simulink model "FilterLib_Test"  (R2018a)
settings: Solver=FixedStepDiscrete  StartTime=0.0  StopTime=5  FixedStep=Ts_task  RelTol=1e-3
PreLoadFcn:
  | Ts_task = 0.001;
InitFcn:
  | if ~exist('Ts_task','var'), Ts_task = 0.001; end
libraries: FilterLib x4
settings Model: Creator=Ismail Shaikh  LastModifiedBy=Ismail Shaikh

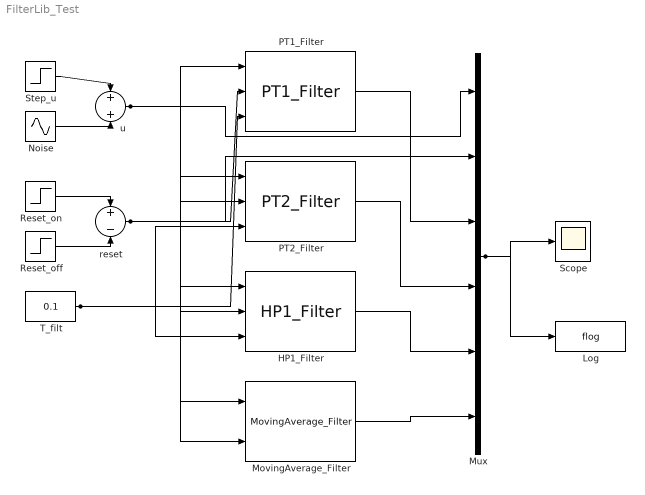
== system FilterLib_Test ==
  HP1_Filter : FilterLib/HP1_Filter  Ts=Ts_task  Method=Exact: K = 1-exp(-Ts/T)  y0=0
      settings: SourceProductName=Filter Library
  Log : ToWorkspace  VariableName=flog  SaveFormat=Structure With Time  SampleTime=-1
  MovingAverage_Filter : FilterLib/MovingAverage_Filter  N=20  y0=0
      settings: SourceProductName=Filter Library
  Mux : Mux  Inputs=6
  Noise : Sin  Amplitude=0.2  Frequency=2*pi*50  SampleTime=Ts_task
  PT1_Filter : FilterLib/PT1_Filter  Ts=Ts_task  Method=Exact: K = 1-exp(-Ts/T)  y0=0
      settings: SourceProductName=Filter Library
  PT2_Filter : FilterLib/PT2_Filter  Ts=Ts_task  Method=Exact: K = 1-exp(-Ts/T)  y0=0
      settings: SourceProductName=Filter Library
  Reset_off : Step  Time=3.05  SampleTime=Ts_task
  Reset_on : Step  Time=3  SampleTime=Ts_task
  Scope : Scope
  Step_u : Step  Time=0.5  SampleTime=Ts_task
  T_filt : Constant  Value=0.1
  reset : Sum  Inputs=+-
  u : Sum
  wires:
  Step_u/1 -> u/1
  Noise/1 -> u/2
  Reset_on/1 -> reset/1
  Reset_off/1 -> reset/2
  u/1 -> PT1_Filter/1, PT2_Filter/1, HP1_Filter/1, MovingAverage_Filter/1, Mux/1
  reset/1 -> PT1_Filter/2, PT2_Filter/2, HP1_Filter/2, MovingAverage_Filter/2, Mux/2
  T_filt/1 -> PT1_Filter/3, PT2_Filter/3, HP1_Filter/3
  PT1_Filter/1 -> Mux/3
  PT2_Filter/1 -> Mux/4
  HP1_Filter/1 -> Mux/5
  MovingAverage_Filter/1 -> Mux/6
  Mux/1 -> Scope/1, Log/1
